simulink model "reduce_emf_before_speedloop"  (R2024b)
settings: Solver=FixedStepAuto  StartTime=0.0  StopTime=25  FixedStep=Tsim  RelTol=1e-4  EnableMultiTasking=on
InitFcn:
  | clc;
  | clear;
  | %% Parameters of the motor
  | Tsim = 1e-6;
  | Tpwm=1e-4;
  | Ts = 1e-4;
  | R = 1.8665;
  | Rs=1.8665;
  | Ls=8.96e-3;
  | Ld = 8.96e-3;
  | Lq = 8.96e-3;
  | L1=(Ld +Lq )/2;
  | L2=(Lq -Ld )/2;
  | flux = 0.21;
  | F=0.00008;
  | J=0.003;
  | Np=4;
  | fpwm = 10e3;
  | Vdc=311;
  | wn=100;
  | %% Controller limiter                                                           % Maximum torque (Nm)
  | I_max = 7.5;                                                    % Maximum current (A)
  | V_max = Vdc/sqrt(3);
  | 
  | 
  | %% 转速环电流环带宽
  | wspd=20;
  | wcur=500;
  | 
  | %% LESO
  | w0=10000;
  | beta1=2*w0-R/Ld;
  | beta2=w0*w0;
  | %% IF启动
  | Iq_if=7;
  | we_if_acc=300;
  | we_if_max=180;
  | we_switch=150;
model workspace (MAT data in the model file):
  new = 0
undefined symbols (not defined in the file or in its folder): DiscIntNeverNeededParam
libraries: spsDCVoltageSourceLib x1, spsGroundLib x1, spsPermanentMagnetSynchronousMachineLib x1, simulink x1, spsUniversalBridgeLib x1, spspowerguiLib x1
(part 2 of 2)

== matlab function reduce_emf_before_speedloop/锁相环1/MATLAB Function ==
  settings: updateMethod=DISCRETE  sampleTime=1e-4
  data: Ed_hat input size=1; Eq_hat input size=1; theta output size=1; we output size=1; IF_sensorless_mode input; id_offset output; vfl_state output; sample_ack input
function [theta,we,id_offset,vfl_state] = fcn(Ed_hat,Eq_hat,IF_sensorless_mode,sample_ack)
%#codegen
%==================================================
% 文档式(12.7)、图12.2：反电动势相位误差 -> PI -> 角度积分。
% Ed_hat、eb端口现在分别接Ed_hat、Eq_hat，单位V，不再接磁链。
% 加入文献12.4.1的虚拟反电动势注入与六段采样状态机。
% 保留原有I/F切换输入及四路输出，外围控制连接保持完整。
%==================================================
persistent theta_z speed_i state tick stable amp
if isempty(theta_z)
    theta_z = 0;
    speed_i = 0;
    state=0; tick=0; stable=0; amp=0;
end
if ~isfinite(Ed_hat) || ~isfinite(Eq_hat) || ~isfinite(IF_sensorless_mode)
    Ed_hat=0; Eq_hat=0; IF_sensorless_mode=0;
end
Ts = 1e-4;                    % 原控制周期，s
wn = 50;                      % PLL带宽初值，rad/s；沿用原代码数值
kp = 2*0.707*wn;              % PI比例增益
ki = wn*wn;                   % PI积分增益
we_max = 1256;                % 原电角速度限幅，rad/s
E_min = 1e-3;                 % 反电动势不足时不更新相位误差，V

% 状态输出与采集函数共用同一控制周期；1表示已切换至无感控制。
% 虚拟电压仅加到PLL使用的Ed，不直接叠加到电机电压命令。
id_offset=0; injection=0;
if IF_sensorless_mode<0.5 || ~isfinite(Ed_hat+Eq_hat)
    state=0; tick=0; stable=0;
end
if state>0
    tick=tick+1;
    % 调试版每个采样阶段固定0.6秒；不等待稳态、工作点或条件数验收。
    % 确认口只保留非有限输入时的数值错误中止，不接受质量门限中止。
    if state>=2 && state<=8 && sample_ack<0
        state=10; tick=0;
    elseif state==5 && tick>7000
        state=6; tick=1;
        amp=min(0.6,max(0.2,0.01*abs(Eq_hat)));
    elseif state>=2 && state<=8 && state~=5 && tick>6000
        state=state+1; tick=1;
    end
    if state>=5 && state<=8, id_offset=-1.0; end
    if state==3 || state==7, injection=amp;
    elseif state==4 || state==8, injection=-amp;
    end
end
vfl_state=int32(state);
Ed_pll=Ed_hat+injection;

% 文档式(12.7)，严格保留atan比值的正负转速语义。
% 分母正则化只用于避免Eq=0数值除零，不改为磁链q轴误差。
if Ed_hat*Ed_hat+Eq_hat*Eq_hat>E_min*E_min
    eq_safe = Eq_hat;
    if abs(eq_safe)<1e-6
        if eq_safe>=0
            eq_safe = 1e-6;
        else
            eq_safe = -1e-6;
        end
    end
    phase_error = atan(-Ed_pll/eq_safe);
else
    phase_error = 0;
end

% PI输出电角速度；限幅饱和时采用条件积分抑制积分累积。
we_unsat = speed_i+kp*phase_error;
we = min(max(we_unsat,-we_max),we_max);
if (we_unsat<=we_max && we_unsat>=-we_max) || ...
   (we_unsat>we_max && phase_error<0) || ...
   (we_unsat< -we_max && phase_error>0)
    speed_i = speed_i+ki*Ts*phase_error;
end
speed_i = min(max(speed_i,-we_max),we_max);

% 输出本周期角度，再以同周期速度推进下一拍角度。
% 外部一拍角度反馈和一拍速度反馈，避免代数环并保持采样对齐。
theta = theta_z;
theta_z = mod(theta_z+Ts*we,2*pi);
% 原有I/F切换至无感0.5秒后开始实验，不再增加相位、速度趋势验收。
% 此处触发的状态转换从下一拍输出，保持注入与状态标记一致。
if state==0 && IF_sensorless_mode>=0.5
    stable=stable+1;
    if stable>=5000
        state=2; tick=0; stable=0;
        amp=min(0.6,max(0.2,0.01*abs(Eq_hat)));
    end
elseif state==0
    stable=0;
end
% 状态9计算结果、状态10中止实验，二者均恢复Id指令偏移和虚拟注入为0。
end

== matlab function reduce_emf_before_speedloop/反电动势观测器 ==
  data: ua input; Ed_hat output; ub input; ia input; ib input; Eq_hat output; we input; theta_hat output; we_out output; theta_z1 input
function [Ed_hat,Eq_hat,theta_hat,we_out] = fcn_improved_paper_strict(ua,ub,ia,ib,we,theta_z1)
%#codegen
%==================================================
% 文档式(12.5)、(12.6)及图12.2：dq降阶扩展反电动势观测器。
% 当前对象为SPMSM，Ld=Lq=Ls，扩展反电动势即永磁体反电动势。
% 输入ua/ub、ia/ib为alpha-beta电压和电流，we为延迟一拍的PLL电角速度。
% theta_z1为延迟一拍的PLL角度，先按同一拍we推进至当前时刻。
% 输出Ed_hat/Eq_hat单位V，直接送入反电动势PLL，不再转换成磁链。
%==================================================
persistent zd zq bd_old bq_old
Ts = 1e-4;                    % 原模型控制周期，s
Ls = 8.96e-3;                 % 参考电感，H
Rs = 1.8665;                  % 参考电阻，ohm
Gr = 500;                     % 所选观测器增益初值，rad/s；文档未给定数值

% 将延迟角度推进一拍，与本周期电压、电流对齐。
theta_c = mod(theta_z1+Ts*we,2*pi);
cs = cos(theta_c);
sn = sin(theta_c);
ud =  cs*ua+sn*ub;
uq = -sn*ua+cs*ub;
id =  cs*ia+sn*ib;
iq = -sn*ia+cs*ib;

% 文档式(12.6)的解耦电压。
ud1 = ud+we*Ls*iq;
uq1 = uq-we*Ls*id;

% 图12.2的降阶实现：
% E_hat = Gr/(s+Gr) * (u_dq1-Rs*i_dq-Ls*p*i_dq)。
% 定义z=E_hat+Gr*Ls*i，消除显式电流微分：
% z_dot=-Gr*z+Gr*(u_dq1+(Gr*Ls-Rs)*i_dq)。
% 两个轴独立，采用梯形法离散，保持100us控制周期。
bd = Gr*(ud1+(Gr*Ls-Rs)*id);
bq = Gr*(uq1+(Gr*Ls-Rs)*iq);
if isempty(zd)
    zd = Gr*Ls*id;            % 初始Ed_hat=0
    zq = Gr*Ls*iq;            % 初始Eq_hat=0
    bd_old = bd;
    bq_old = bq;
else
    a = 0.5*Ts*Gr;
    zd = ((1-a)*zd+0.5*Ts*(bd+bd_old))/(1+a);
    zq = ((1-a)*zq+0.5*Ts*(bq+bq_old))/(1+a);
    bd_old = bd;
    bq_old = bq;
end
Ed_hat = zd-Gr*Ls*id;
Eq_hat = zq-Gr*Ls*iq;

% 辅助监测输出，主闭环只使用前两路反电动势。
if abs(Ed_hat)+abs(Eq_hat)>1e-6
    eq_safe = Eq_hat;
    if abs(eq_safe)<1e-6
        if eq_safe>=0
            eq_safe=1e-6;
        else
            eq_safe=-1e-6;
        end
    end
    theta_hat = mod(theta_c+atan(-Ed_hat/eq_safe),2*pi);
else
    theta_hat = theta_c;
end
we_out = we;
end
